simulink model "Surface_Actuator"  (R2024a)
settings: Solver=FixedStepDiscrete  StartTime=0.0  StopTime=8  FixedStep=0.001  RelTol=1e-3
settings Model: Creator=zz  LastModifiedBy=zz

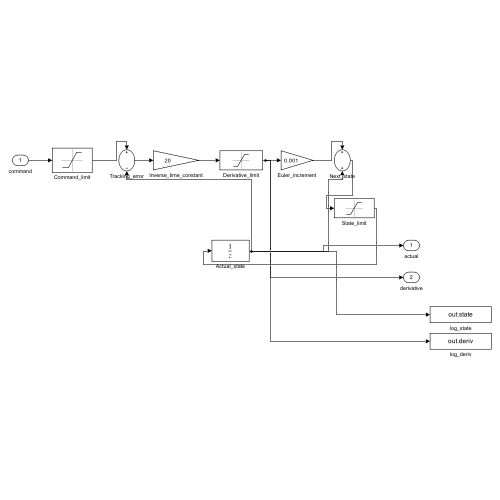
[thumbnail: Simulink's stored preview of the top-level diagram]
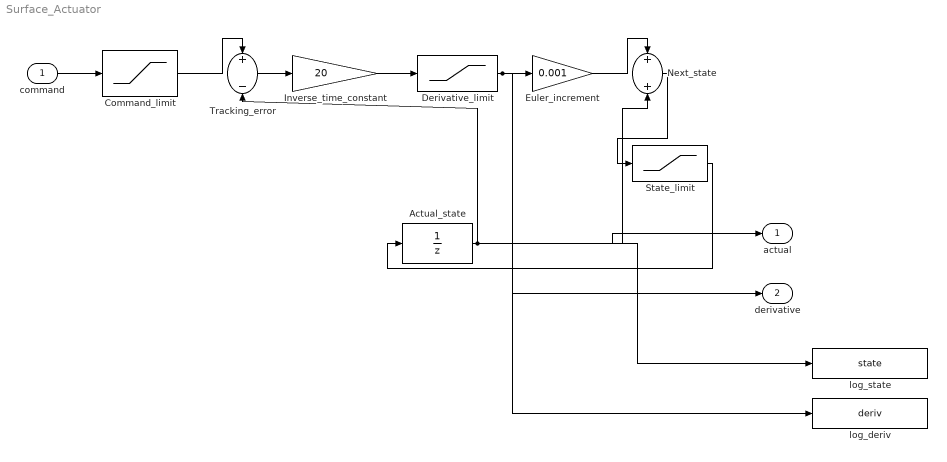
== system Surface_Actuator ==
  command : Inport  PortDimensions=3  SampleTime=0.001
  Actual_state : UnitDelay  InitialCondition=[0;0;0]  SampleTime=0.001
  Command_limit : Saturate  UpperLimit=[0.436332312998582;0.349065850398866;0.349065850398866]  LowerLimit=[-0.436332312998582;-0.349065850398866;-0.349065850398866]
  Derivative_limit : Saturate  UpperLimit=[1.0471975511966;1.0471975511966;1.0471975511966]  LowerLimit=[-1.0471975511966;-1.0471975511966;-1.0471975511966]
  Euler_increment : Gain  Gain=0.001
  Inverse_time_constant : Gain  Gain=20
  Next_state : Sum
  State_limit : Saturate  UpperLimit=[0.436332312998582;0.349065850398866;0.349065850398866]  LowerLimit=[-0.436332312998582;-0.349065850398866;-0.349065850398866]
  Tracking_error : Sum  Inputs=+-
  log_deriv : ToWorkspace  VariableName=deriv  SaveFormat=Timeseries
  log_state : ToWorkspace  VariableName=state  SaveFormat=Timeseries
  actual : Outport
  derivative : Outport  Port=2
  wires:
  command/1 -> Command_limit/1
  Command_limit/1 -> Tracking_error/1
  Actual_state/1 -> Tracking_error/2, Next_state/2, actual/1, log_state/1
  Tracking_error/1 -> Inverse_time_constant/1
  Inverse_time_constant/1 -> Derivative_limit/1
  Derivative_limit/1 -> Euler_increment/1, derivative/1, log_deriv/1
  Euler_increment/1 -> Next_state/1
  Next_state/1 -> State_limit/1
  State_limit/1 -> Actual_state/1
